simulink model "rcrc_sim"  (R2024a)
settings: Solver=ode23tb  StartTime=0.0  StopTime=0.1  RelTol=1e-3
values from neighbouring files (symbols this model uses):
  C1 = 470e-9    (= 4.7e-07)    [rcrc_ini.m]
  C2 = C1    (= 4.7e-07)    [rcrc_ini.m]
  R1 = 4.7e3    (= 4700)    [rcrc_ini.m]
  R2 = R1    (= 4700)    [rcrc_ini.m]
settings Model: Creator=pmic  LastModifiedBy=pichim
settings SolverCC: AlgebraicLoopSolver=TrustRegion
settings DebuggingCC: UnconnectedInputMsg=warning  UnconnectedOutputMsg=warning  UnconnectedLineMsg=warning
settings ModelReferenceCC: EnableRefExpFcnMdlSchedulingChecks=on
settings RTWCC: GPUComputeCapability=3.5  DLArmComputeVersion=19.05

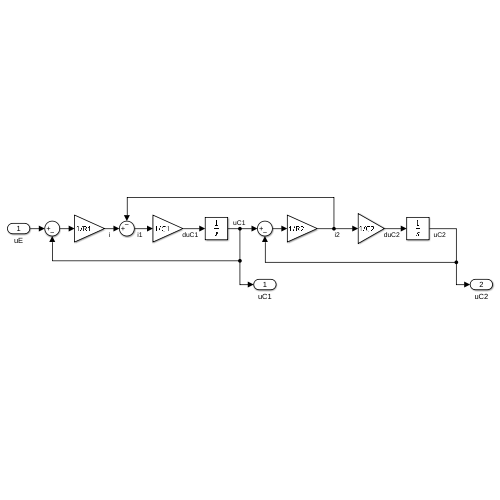
[thumbnail: Simulink's stored preview of the top-level diagram]
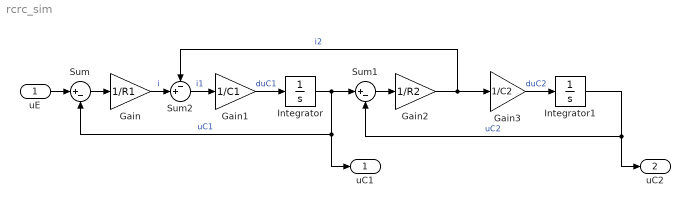
== system rcrc_sim ==
  uE : Inport
  Gain : Gain  Gain=1/R1
  Gain1 : Gain  Gain=1/C1
  Gain2 : Gain  Gain=1/R2
  Gain3 : Gain  Gain=1/C2
  Integrator : Integrator
  Integrator1 : Integrator
  Sum : Sum  Inputs=|+-
  Sum1 : Sum  Inputs=|+-
  Sum2 : Sum  Inputs=-+|
  uC1 : Outport
  uC2 : Outport  Port=2
  wires:
  Gain3/1 -> Integrator1/1  "duC2"
  Sum/1 -> Gain/1
  Integrator/1 -> uC1/1, Sum/2, Sum1/1  "uC1"
  Gain1/1 -> Integrator/1  "duC1"
  Integrator1/1 -> uC2/1, Sum1/2  "uC2"
  Sum2/1 -> Gain1/1  "i1"
  Gain/1 -> Sum2/2  "i"
  Sum1/1 -> Gain2/1
  Gain2/1 -> Gain3/1, Sum2/1  "i2"
  uE/1 -> Sum/1
